simulink model "big_brain"  (R2026b)
settings: Solver=VariableStepAuto  StopTime=50
undefined symbols (not defined in the file): max_acceleration, max_speed
settings Model: DataDictionary=Acc_data.sldd  Creator=_The_FooL  LastModifiedBy=_The_FooL

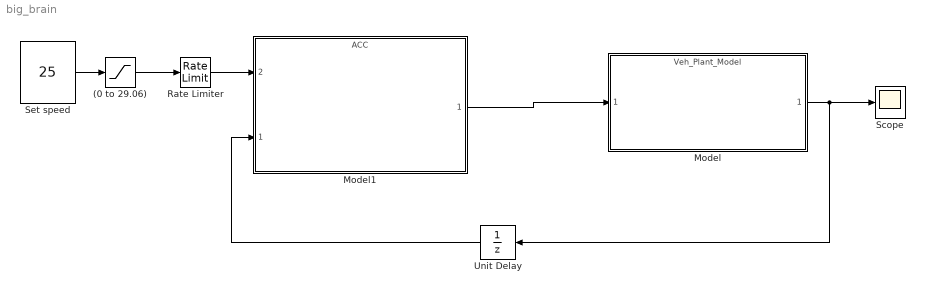
== system big_brain ==
  (0 to 29.06) : Saturate  UpperLimit=max_speed  LowerLimit=0
  Model : ModelReference  ModelNameDialog=Veh_Plant_Model.slx  SimulationMode=Normal  ModelReferenceVersion=1.5
  Model1 : ModelReference  ModelNameDialog=ACC.slx  SimulationMode=Normal  ModelReferenceVersion=1.4
      settings: PortSchema="{\"entries\":[{\"content\":{\"sides\":[{\"content\":{\"connectorIds\":[\"In2\",\"In1\"]},\"type\":\"ConnectorPlacement.EquallySpacedRectSide\",\"uuid\":\"be300e41-5095-4600-bc3d-09b0a62efb9b\"},{\"content\":{\"connectorIds\":[\"Out1\"],\"side\":\"RIGHT\"},\"type\":\"ConnectorPlacement.EquallySpacedRectSide\",\"uuid\":\"fe44e470-adb8-4a91-807d-ef1b51409f62\"},{\"content\":{\"side\":\"TOP\"},\"type\":\"ConnectorPlacement.EquallySpacedRectSide\",\"uuid\":\"d20f43b2-a0b1-4ff2-a577-7ac1638984f0\"}]},\"type\":\"ConnectorPlacement.EquallySpacedConnector\",\"uuid\":\"cabc0c71-e9f8-439c-bc50-6f2c107042d1\"}],\"packageUris\":[\"http://schema.mathworks.com/mf0/Connector/R2020b\"],\"version\":\"1.0\"}"
  Rate Limiter : RateLimiter  RisingSlewLimit=max_acceleration  FallingSlewLimit=-max_acceleration  SampleTimeMode=inherited
  Scope : Scope
      settings: ActiveDisplayYMinimum=-17.198369468834134  ActiveDisplayYMaximum=83.3131920634534
  Set speed : Constant  Value=25
  Unit Delay : UnitDelay  SampleTime=-1
  wires:
  Model1/1 -> Model/1
  Set speed/1 -> (0 to 29.06)/1
  Model/1 -> Scope/1, Unit Delay/1
  Unit Delay/1 -> Model1/1
  (0 to 29.06)/1 -> Rate Limiter/1
  Rate Limiter/1 -> Model1/2
